simulink model "DynKynValidation"  (R2026b)
settings: Solver=ode5  StopTime=6049.5  FixedStep=1
values from neighbouring files (symbols this model uses):
  A_surf = [Ly*Lz; Lx*Lz; Lx*Ly; Ly*Lz; Lx*Lz; Lx*Ly;            A_panel; A_panel; A_panel; A_panel]    [ValidationAirDrag.m]
  e = e0    (= 0.001)    [ValidationAirDrag.m]    (also in max_disturbance.m = 0.0011)
  i_inc = deg2rad(97.7)    [ValidationAirDrag.m]
  n = sqrt(mu_earth/R^3)    [ValidationAirDrag.m]
  N_surf = [1 0 0; 0 1 0; 0 0 1; -1 0 0; 0 -1 0; 0 0 -1;            1 0 0; -1 0 0; 1 0 0; -1 0 0]    [ValidationAirDrag.m]
  r_CM = r_CM0    [ValidationAirDrag.m]
  R_CP_geom = [Lx/2 0 0; 0 Ly/2 0; 0 0 Lz/2;              -Lx/2 0 0; 0 -Ly/2 0; 0 0 -Lz/2;               0 d_panel 0; 0 d_panel 0; 0 -d_panel 0; 0 -d_panel 0]'    [ValidationAirDrag.m]
undefined symbols (not defined in the file or in its folder): a, angles0, Cd, ecc, hr, I, I_inv, incl, J, rho_atm, true_anomaly_0, w_earth, wB0
libraries: matrix_library x2
settings Model: Creator=39333  LastModifiedBy=enea

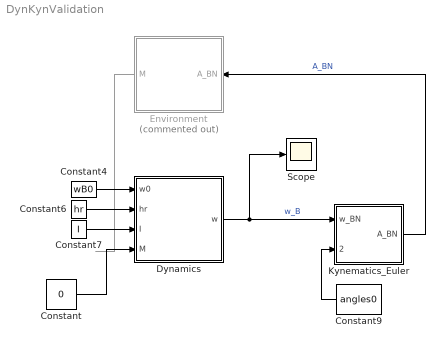
== system DynKynValidation ==
  Constant : Constant  Value=0
  Constant4 : Constant  Value=wB0
  Constant6 : Constant  Value=hr
  Constant7 : Constant  Value=I
  Constant9 : Constant  Value=angles0
  Dynamics : Subsystem
  Environment : Subsystem  Commented=on
  Kynematics_Euler : Subsystem
  Scope : Scope
      settings: ActiveDisplayYMinimum=-0.28630791111671289  ActiveDisplayYMaximum=1.1434373830960349  DataLoggingVariableName=ScopeData2
  wires:
  Constant9/1 -> Kynematics_Euler/2(angles0)
  Kynematics_Euler/1(A_BN) -> Environment/1(A_BN)  "A_BN"
  Environment/1(M) -> ?
  Constant7/1 -> Dynamics/3(I)
  Constant6/1 -> Dynamics/2(hr)
  Constant/1 -> Dynamics/4(M)
  Constant4/1 -> Dynamics/1(w0)
  Dynamics/1(w) -> Scope/1, Kynematics_Euler/1(w_BN)  "w_B"

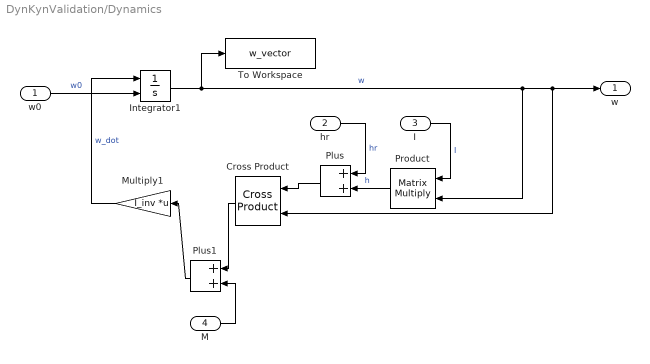
== system DynKynValidation/Dynamics ==
  w0 : Inport
  hr : Inport  Port=2
  I : Inport  Port=3
  M : Inport  Port=4
  Cross Product : matrix_library/Cross Product
  Integrator1 : Integrator  InitialConditionSource=external
  Multiply1 : Gain  Gain=I_inv  Multiplication=Matrix(K*u)
  Plus : Sum
  Plus1 : Sum
  Product : Product  Multiplication=Matrix(*)
  To Workspace : ToWorkspace  VariableName=w_vector  SampleTime=-1
  w : Outport
  wires:
  M/1 -> Plus1/2
  Plus1/1 -> Multiply1/1
  Cross Product/1 -> Plus1/1
  Multiply1/1 -> Integrator1/1  "w_dot"
  I/1 -> Product/1  "I"
  Plus/1 -> Cross Product/1
  Product/1 -> Plus/2  "h"
  Integrator1/1 -> Product/2, Cross Product/2, w/1, To Workspace/1  "w"
  w0/1 -> Integrator1/2  "w0"
  hr/1 -> Plus/1  "hr"

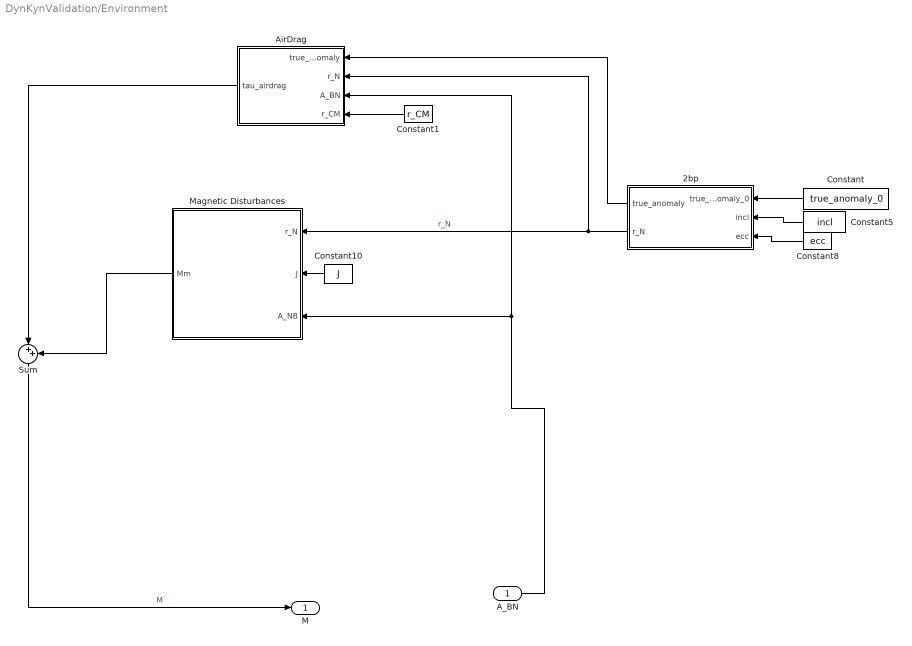
== system DynKynValidation/Environment ==
  A_BN : Inport
  2bp : Subsystem
  AirDrag : Subsystem
  Constant : Constant  Value=true_anomaly_0
  Constant1 : Constant  Value=r_CM
  Constant10 : Constant  Value=J
  Constant5 : Constant  Value=incl
  Constant8 : Constant  Value=ecc
  Magnetic Disturbances : Subsystem
  Sum : Sum  Inputs=|++
  M : Outport
  wires:
  2bp/2(r_N) -> AirDrag/2(r_N), Magnetic Disturbances/1(r_N)  "r_N"
  Magnetic Disturbances/1(Mm) -> Sum/2
  Constant1/1 -> AirDrag/4(r_CM)
  AirDrag/1(tau_airdrag) -> Sum/1
  Constant/1 -> 2bp/1(true_anomaly_0)
  2bp/1(true_anomaly) -> AirDrag/1(true_anomaly)
  Constant5/1 -> 2bp/2(incl)
  Constant10/1 -> Magnetic Disturbances/2(J)
  Constant8/1 -> 2bp/3(ecc)
  A_BN/1 -> AirDrag/3(A_BN), Magnetic Disturbances/3(A_NB)
  Sum/1 -> M/1  "M"

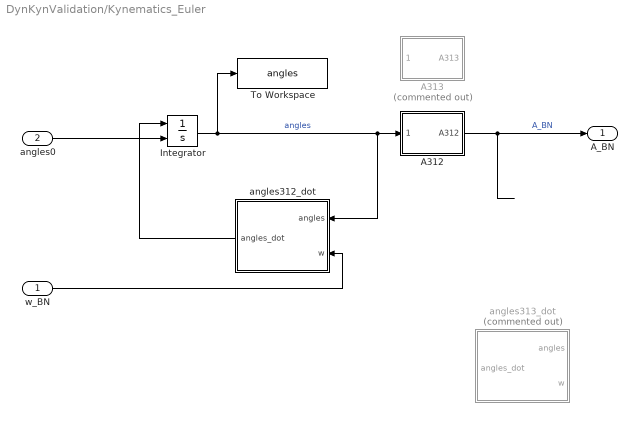
== system DynKynValidation/Kynematics_Euler ==
  w_BN : Inport
  angles0 : Inport  Port=2
  A312 : Subsystem
  A313 : Subsystem  Commented=on
  Integrator : Integrator  InitialConditionSource=external
  To Workspace : ToWorkspace  VariableName=angles  SampleTime=-1
  angles312_dot : Subsystem
  angles313_dot : Subsystem  Commented=on
  A_BN : Outport
  wires:
  Integrator/1 -> A312/1(angles), angles312_dot/1(angles), To Workspace/1  "angles"
  A312/1(A312) -> A_BN/1  "A_BN"
  angles0/1 -> Integrator/2
  angles312_dot/1(angles_dot) -> Integrator/1
  w_BN/1 -> angles312_dot/2(w)

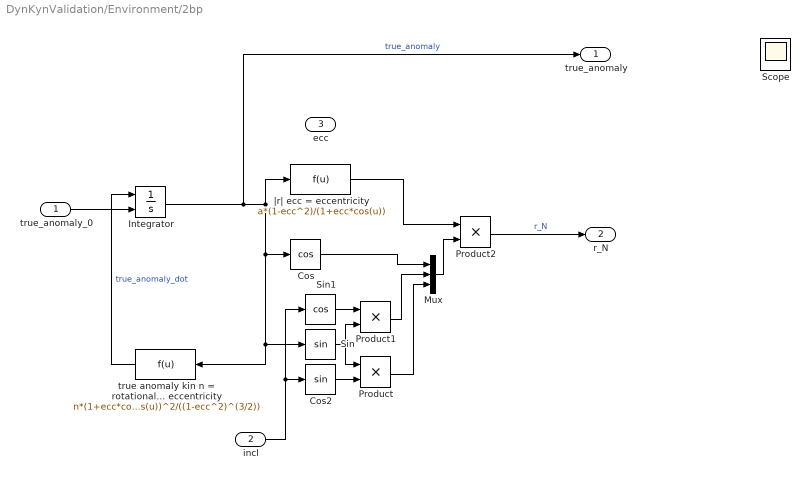
== system DynKynValidation/Environment/2bp ==
  true_anomaly_0 : Inport
  incl : Inport  Port=2
  ecc : Inport  Port=3
  Cos : Trigonometry  Operator=cos
  Cos2 : Trigonometry
  Integrator : Integrator  InitialConditionSource=external
  Mux : Mux  Inputs=3
  Product : Product
  Product1 : Product
  Product2 : Product
  Scope : Scope
  Sin : Trigonometry
  Sin1 : Trigonometry  Operator=cos
  "true anomaly kin n = rotational rate ecc = eccentricity " : Fcn  Expr=n*(1+ecc*cos(u))^2/((1-ecc^2)^(3/2))
  |r| ecc = eccentricity : Fcn  Expr=a*(1-ecc^2)/(1+ecc*cos(u))
  true_anomaly : Outport
  r_N : Outport  Port=2
  wires:
  Sin1/1 -> Product1/1
  Product/1 -> Mux/3
  |r| ecc = eccentricity/1 -> Product2/1
  Cos/1 -> Mux/1
  Product1/1 -> Mux/2
  Integrator/1 -> true_anomaly/1, |r| ecc = eccentricity/1, Sin/1, "true anomaly kin n = rotational rate ecc = eccentricity "/1, Cos/1  "true_anomaly"
  Mux/1 -> Product2/2
  Product2/1 -> r_N/1  "r_N"
  Sin/1 -> Product1/2, Product/1
  "true anomaly kin n = rotational rate ecc = eccentricity "/1 -> Integrator/1  "true_anomaly_dot"
  true_anomaly_0/1 -> Integrator/2
  incl/1 -> Cos2/1, Sin1/1
  Cos2/1 -> Product/2

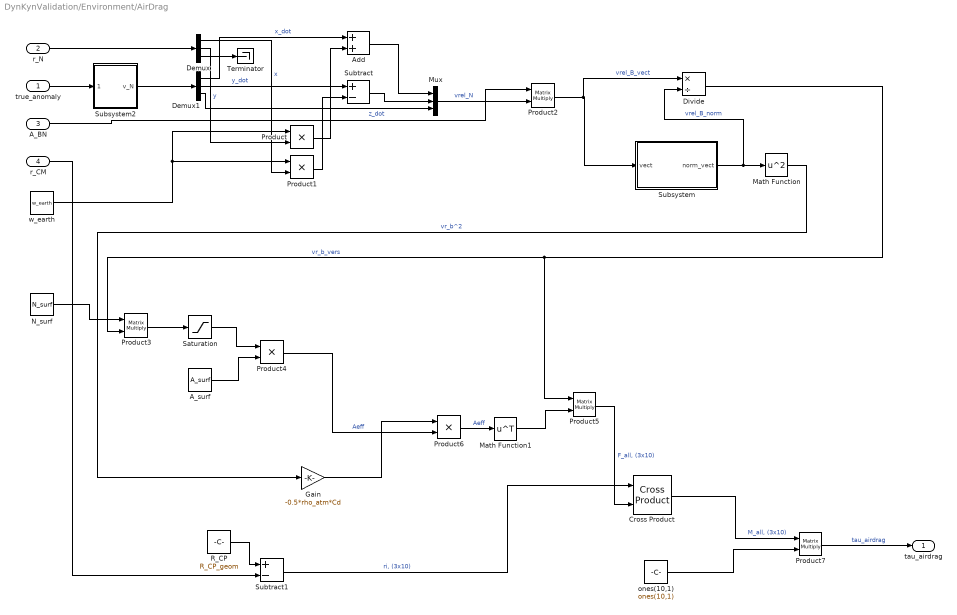
== system DynKynValidation/Environment/AirDrag ==
  true_anomaly : Inport
  r_N : Inport  Port=2
  A_BN : Inport  Port=3
  r_CM : Inport  Port=4
  A_surf : Constant  Value=A_surf
  Add : Sum
  Cross Product : matrix_library/Cross Product
  Demux : Demux  Outputs=3
  Demux1 : Demux  Outputs=3
  Divide : Product  Inputs=*/
  Gain : Gain  Gain=-0.5*rho_atm*Cd
  Math Function : Math  Operator=square
  Math Function1 : Math  Operator=transpose
  Mux : Mux  Inputs=3
  N_surf : Constant  Value=N_surf
  Product{,1,4,6} (4 alike) : Product
  Product{2..3,5,7} (4 alike) : Product  Multiplication=Matrix(*)
  R_CP : Constant  Value=R_CP_geom
  Saturation : Saturate  UpperLimit=inf  LowerLimit=0
  Subsystem : Subsystem
  Subsystem2 : Subsystem
  Subtract : Sum  Inputs=+-
  Subtract1 : Sum  Inputs=+-
  Terminator : Terminator
  ones(10,1) : Constant  Value=ones(10,1)
  w_earth : Constant  Value=w_earth
  tau_airdrag : Outport
  wires:
  Divide/1 -> Product3/2, Product5/1  "vr_b_vers"
  Product4/1 -> Product6/2  "Aeff"
  w_earth/1 -> Product/1, Product1/1
  Demux/3 -> Terminator/1
  Math Function1/1 -> Product5/2
  Demux/2 -> Product/2  "y"
  Demux1/2 -> Subtract/1  "y_dot"
  Demux/1 -> Product1/2  "x"
  Product6/1 -> Math Function1/1  "Aeff"
  Product2/1 -> Divide/1, Subsystem/1(vect)  "vrel_B_vect"
  Gain/1 -> Product6/1
  Add/1 -> Mux/1
  Cross Product/1 -> Product7/1  "M_all, (3x10)"
  Demux1/1 -> Add/1  "x_dot"
  Subsystem2/1(v_N) -> Demux1/1
  Subsystem/1(norm_vect) -> Divide/2, Math Function/1  "vrel_B_norm"
  A_surf/1 -> Product4/2
  Subtract/1 -> Mux/2
  R_CP/1 -> Subtract1/1
  Subtract1/1 -> Cross Product/1  "ri, (3x10)"
  Demux1/3 -> Mux/3  "z_dot"
  Product/1 -> Add/2
  Mux/1 -> Product2/2  "vrel_N"
  Product3/1 -> Saturation/1
  Saturation/1 -> Product4/1
  A_BN/1 -> Product2/1
  Math Function/1 -> Gain/1  "vr_b^2"
  Product1/1 -> Subtract/2
  N_surf/1 -> Product3/1
  Product7/1 -> tau_airdrag/1  "tau_airdrag"
  ones(10,1)/1 -> Product7/2
  Product5/1 -> Cross Product/2  "F_all, (3x10)"
  r_N/1 -> Demux/1
  true_anomaly/1 -> Subsystem2/1(true_anomaly)
  r_CM/1 -> Subtract1/2

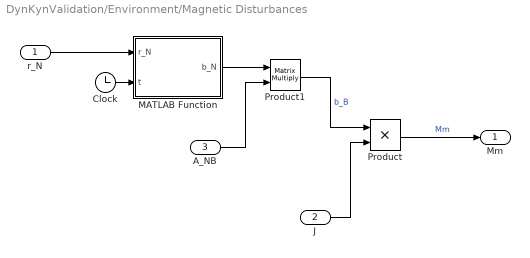
== system DynKynValidation/Environment/Magnetic Disturbances ==
  r_N : Inport
  J : Inport  Port=2
  A_NB : Inport  Port=3
  Clock : Clock
  MATLAB Function : MATLAB Function  TreatAsAtomicUnit=on
  Product : Product
  Product1 : Product  Multiplication=Matrix(*)
  Mm : Outport
  wires:
  Product1/1 -> Product/1  "b_B"
  Clock/1 -> MATLAB Function/2(t)
  MATLAB Function/1(b_N) -> Product1/1
  Product/1 -> Mm/1  "Mm"
  A_NB/1 -> Product1/2
  J/1 -> Product/2
  r_N/1 -> MATLAB Function/1(r_N)

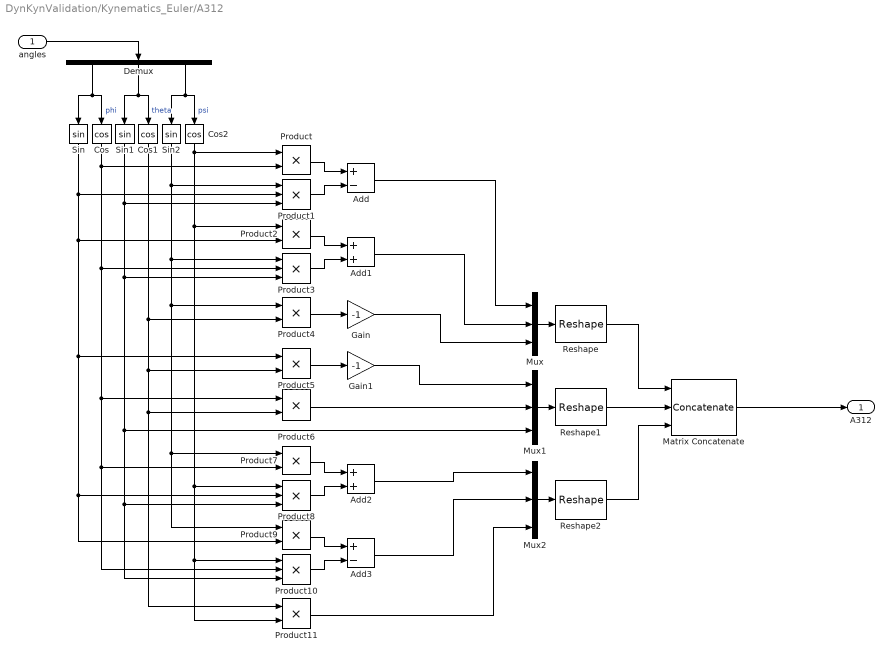
== system DynKynValidation/Kynematics_Euler/A312 ==
  angles : Inport
  Add : Sum  Inputs=+-
  Add1 : Sum
  Add2 : Sum
  Add3 : Sum  Inputs=+-
  Cos : Trigonometry  Operator=cos
  Cos1 : Trigonometry  Operator=cos
  Cos2 : Trigonometry  Operator=cos
  Demux : Demux  Outputs=3
  Gain : Gain  Gain=-1
  Gain1 : Gain  Gain=-1
  Matrix Concatenate : Concatenate  NumInputs=3  Mode=Multidimensional array
  Mux : Mux  Inputs=3
  Mux1 : Mux  Inputs=3
  Mux2 : Mux  Inputs=3
  Product{,2,4..7,9,11} (8 alike) : Product
  Product{1,3,8,10} (4 alike) : Product  Inputs=3
  Reshape : Reshape  OutputDimensionality=Row vector (2-D)  OutputDimensions=[3,1]
  Reshape1 : Reshape  OutputDimensionality=Row vector (2-D)  OutputDimensions=[3,1]
  Reshape2 : Reshape  OutputDimensionality=Row vector (2-D)  OutputDimensions=[3,1]
  Sin : Trigonometry
  Sin1 : Trigonometry
  Sin2 : Trigonometry
  A312 : Outport
  wires:
  Add3/1 -> Mux2/2
  Sin/1 -> Product2/2, Product9/2, Product8/2, Product5/1, Product1/2
  Add1/1 -> Mux/2
  Demux/2 -> Cos1/1, Sin1/1  "theta"
  Sin1/1 -> Product10/3, Product8/3, Mux1/3, Product3/3, Product1/3
  Cos2/1 -> Product2/1, Product11/2, Product10/1, Product8/1, Product/1
  Demux/1 -> Cos/1, Sin/1  "phi"
  Cos1/1 -> Product5/2, Product11/1, Product6/2, Product4/2
  Product/1 -> Add/1
  Sin2/1 -> Product4/1, Product7/1, Product9/1, Product3/1, Product1/1
  Gain1/1 -> Mux1/1
  Product4/1 -> Gain/1
  Product11/1 -> Mux2/3
  Cos/1 -> Product10/2, Product7/2, Product6/1, Product3/2, Product/2
  Demux/3 -> Sin2/1, Cos2/1  "psi"
  Product10/1 -> Add3/2
  Product5/1 -> Gain1/1
  Add2/1 -> Mux2/1
  Product7/1 -> Add2/1
  Product3/1 -> Add1/2
  Product8/1 -> Add2/2
  Product9/1 -> Add3/1
  Product1/1 -> Add/2
  Reshape/1 -> Matrix Concatenate/1
  Product6/1 -> Mux1/2
  Gain/1 -> Mux/3
  Add/1 -> Mux/1
  Product2/1 -> Add1/1
  Matrix Concatenate/1 -> A312/1
  Mux2/1 -> Reshape2/1
  Reshape2/1 -> Matrix Concatenate/3
  Reshape1/1 -> Matrix Concatenate/2
  Mux/1 -> Reshape/1
  Mux1/1 -> Reshape1/1
  angles/1 -> Demux/1

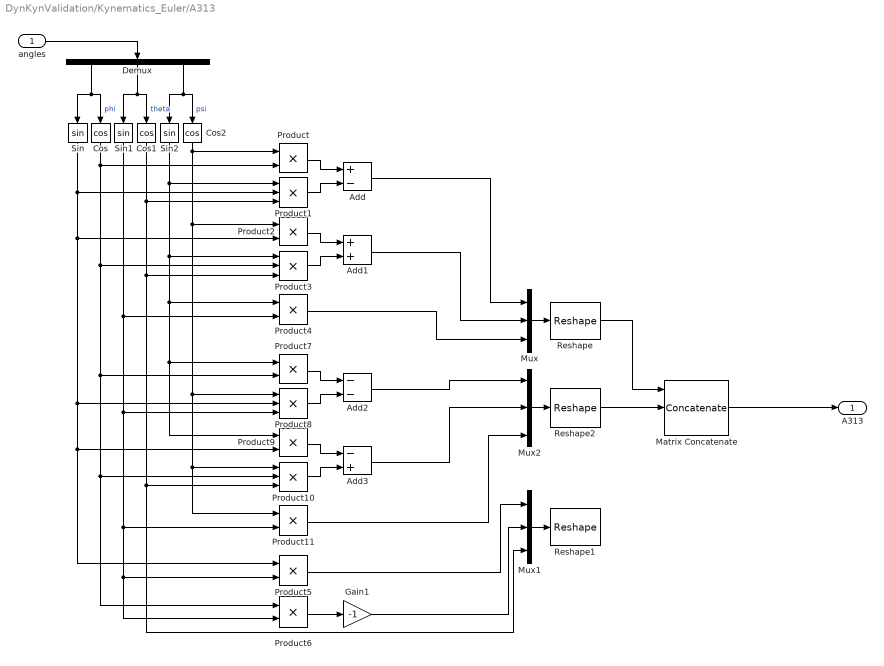
== system DynKynValidation/Kynematics_Euler/A313 ==
  angles : Inport
  Add : Sum  Inputs=+-
  Add1 : Sum
  Add2 : Sum  Inputs=--
  Add3 : Sum  Inputs=-+
  Cos : Trigonometry  Operator=cos
  Cos1 : Trigonometry  Operator=cos
  Cos2 : Trigonometry  Operator=cos
  Demux : Demux  Outputs=3
  Gain1 : Gain  Gain=-1
  Matrix Concatenate : Concatenate  NumInputs=3  Mode=Multidimensional array
  Mux : Mux  Inputs=3
  Mux1 : Mux  Inputs=3
  Mux2 : Mux  Inputs=3
  Product{,2,4..7,9,11} (8 alike) : Product
  Product{1,3,8,10} (4 alike) : Product  Inputs=3
  Reshape : Reshape  OutputDimensionality=Row vector (2-D)  OutputDimensions=[3,1]
  Reshape1 : Reshape  OutputDimensionality=Row vector (2-D)  OutputDimensions=[3,1]
  Reshape2 : Reshape  OutputDimensionality=Row vector (2-D)  OutputDimensions=[3,1]
  Sin : Trigonometry
  Sin1 : Trigonometry
  Sin2 : Trigonometry
  A313 : Outport
  wires:
  Add3/1 -> Mux2/2
  Sin/1 -> Product2/2, Product5/1, Product9/2, Product8/2, Product1/2
  Add1/1 -> Mux/2
  Demux/2 -> Cos1/1, Sin1/1  "theta"
  Sin1/1 -> Product4/2, Product11/2, Product6/2, Product5/2, Product8/3
  Cos2/1 -> Product2/1, Product11/1, Product10/1, Product8/1, Product/1
  Demux/1 -> Cos/1, Sin/1  "phi"
  Cos1/1 -> Product1/3, Product3/3, Mux1/3, Product10/3
  Product/1 -> Add/1
  Sin2/1 -> Product4/1, Product7/1, Product9/1, Product3/1, Product1/1
  Product5/1 -> Mux1/1
  Product11/1 -> Mux2/3
  Cos/1 -> Product6/1, Product10/2, Product7/2, Product3/2, Product/2
  Demux/3 -> Sin2/1, Cos2/1  "psi"
  Product10/1 -> Add3/2
  Add2/1 -> Mux2/1
  Product7/1 -> Add2/1
  Product3/1 -> Add1/2
  Product8/1 -> Add2/2
  Product9/1 -> Add3/1
  Product1/1 -> Add/2
  Reshape/1 -> Matrix Concatenate/1
  Product6/1 -> Gain1/1
  Product4/1 -> Mux/3
  Add/1 -> Mux/1
  Product2/1 -> Add1/1
  Matrix Concatenate/1 -> A313/1
  Mux2/1 -> Reshape2/1
  Mux/1 -> Reshape/1
  Mux1/1 -> Reshape1/1
  angles/1 -> Demux/1
  Reshape2/1 -> Matrix Concatenate/2
  Gain1/1 -> Mux1/2

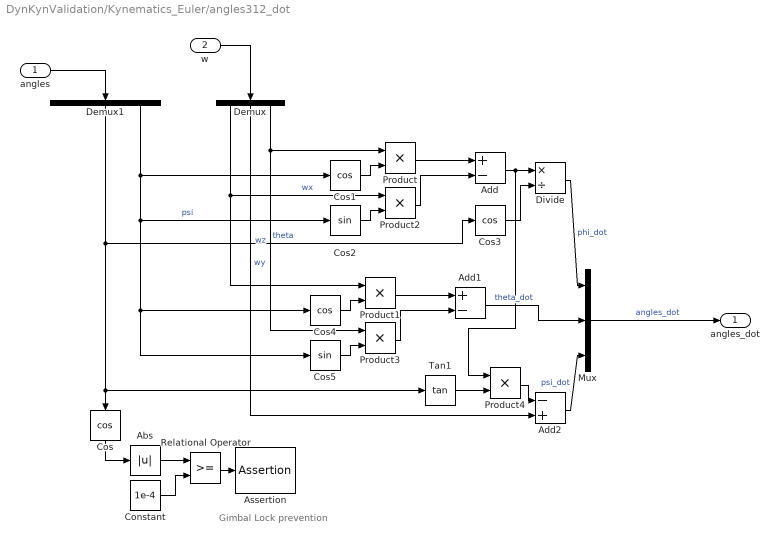
== system DynKynValidation/Kynematics_Euler/angles312_dot ==
  note: Gimbal Lock prevention
  angles : Inport
  w : Inport  Port=2
  Abs : Abs  SaturateOnIntegerOverflow=off
  Add : Sum  Inputs=+-
  Add1 : Sum  Inputs=+-
  Add2 : Sum  Inputs=-+
  Assertion : Assertion  AssertionFailFcn='Gimbal Lock Detected'  StopWhenAssertionFail=off
  Constant : Constant  Value=1e-4
  Cos{,1,3..4} (4 alike) : Trigonometry  Operator=cos
  Cos2 : Trigonometry
  Cos5 : Trigonometry
  Demux : Demux  Outputs=3
  Demux1 : Demux  Outputs=3
  Divide : Product  Inputs=*/
  Mux : Mux  Inputs=3
  Product{,1..4} (5 alike) : Product
  Relational Operator : RelationalOperator  OutDataTypeStr=boolean  RndMeth=Simplest  InputSameDT=off
  Tan1 : Trigonometry  Operator=tan
  angles_dot : Outport
  wires:
  Cos5/1 -> Product3/2
  Add/1 -> Product4/1, Divide/1
  Cos2/1 -> Product2/2
  Demux1/3 -> Cos1/1, Cos2/1, Cos4/1, Cos5/1  "psi"
  Demux1/2 -> Cos/1, Tan1/1, Cos3/1  "theta"
  Cos4/1 -> Product1/2
  Cos1/1 -> Product/2
  Demux/3 -> Product3/1, Product/1  "wz"
  Demux/1 -> Product1/1, Product2/1  "wx"
  Product/1 -> Add/1
  Tan1/1 -> Product4/2
  w/1 -> Demux/1
  Divide/1 -> Mux/1  "phi_dot"
  Cos3/1 -> Divide/2
  Product2/1 -> Add/2
  Product3/1 -> Add1/2
  Product1/1 -> Add1/1
  Add1/1 -> Mux/2  "theta_dot"
  Mux/1 -> angles_dot/1  "angles_dot"
  Product4/1 -> Add2/1
  Add2/1 -> Mux/3  "psi_dot"
  Demux/2 -> Add2/2  "wy"
  angles/1 -> Demux1/1
  Relational Operator/1 -> Assertion/1
  Constant/1 -> Relational Operator/2
  Abs/1 -> Relational Operator/1
  Cos/1 -> Abs/1

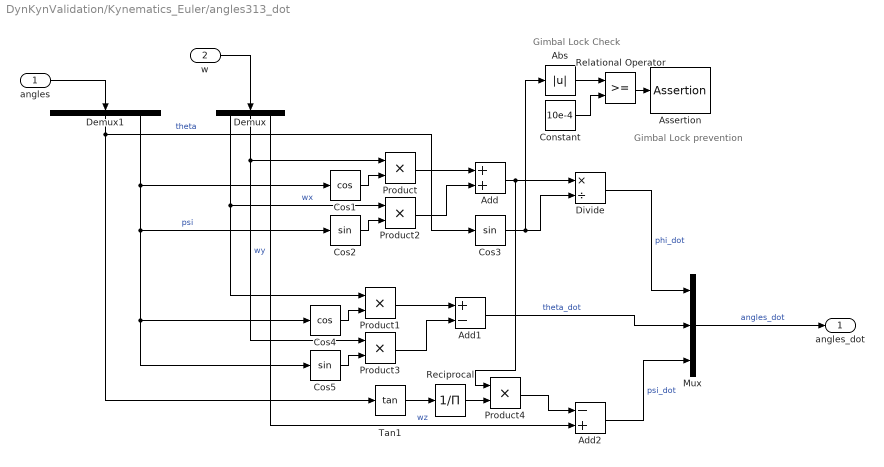
== system DynKynValidation/Kynematics_Euler/angles313_dot ==
  note: Gimbal Lock Check
  note: Gimbal Lock prevention
  angles : Inport
  w : Inport  Port=2
  Abs : Abs  SaturateOnIntegerOverflow=off
  Add : Sum
  Add1 : Sum  Inputs=+-
  Add2 : Sum  Inputs=-+
  Assertion : Assertion  AssertionFailFcn='Gimbal Lock Detected'  StopWhenAssertionFail=off
  Constant : Constant  Value=10e-4
  Cos1 : Trigonometry  Operator=cos
  Cos2 : Trigonometry
  Cos3 : Trigonometry
  Cos4 : Trigonometry  Operator=cos
  Cos5 : Trigonometry
  Demux : Demux  Outputs=3
  Demux1 : Demux  Outputs=3
  Divide : Product  Inputs=*/
  Mux : Mux  Inputs=3
  Product{,1..4} (5 alike) : Product
  Reciprocal : Product  Inputs=/
  Relational Operator : RelationalOperator  OutDataTypeStr=boolean  RndMeth=Simplest  InputSameDT=off
  Tan1 : Trigonometry  Operator=tan
  angles_dot : Outport
  wires:
  Cos5/1 -> Product3/2
  Add/1 -> Product4/1, Divide/1
  Cos2/1 -> Product2/2
  Demux1/3 -> Cos4/1, Cos5/1, Cos2/1, Cos1/1  "psi"
  Demux1/2 -> Tan1/1, Cos3/1  "theta"
  Cos4/1 -> Product1/2
  Cos1/1 -> Product/2
  Demux/1 -> Product1/1, Product2/1  "wx"
  Product/1 -> Add/1
  Tan1/1 -> Reciprocal/1
  w/1 -> Demux/1
  Divide/1 -> Mux/1  "phi_dot"
  Product2/1 -> Add/2
  Product3/1 -> Add1/2
  Product1/1 -> Add1/1
  Add1/1 -> Mux/2  "theta_dot"
  Mux/1 -> angles_dot/1  "angles_dot"
  Product4/1 -> Add2/1
  Add2/1 -> Mux/3  "psi_dot"
  Demux/2 -> Product/1, Product3/1  "wy"
  angles/1 -> Demux1/1
  Demux/3 -> Add2/2  "wz"
  Reciprocal/1 -> Product4/2
  Cos3/1 -> Abs/1, Divide/2
  Relational Operator/1 -> Assertion/1
  Abs/1 -> Relational Operator/1
  Constant/1 -> Relational Operator/2

== system DynKynValidation/Environment/AirDrag/Subsystem ==
  vect : Inport
  Add1 : Sum  Inputs=+++
  Demux2 : Demux  Outputs=3
  Math Function : Math  Operator=square
  Math Function1 : Math  Operator=square
  Math Function2 : Math  Operator=square
  Sqrt : Sqrt
  norm_vect : Outport
  wires:
  Math Function1/1 -> Add1/2
  Math Function2/1 -> Add1/3
  Demux2/2 -> Math Function1/1
  Math Function/1 -> Add1/1
  vect/1 -> Demux2/1
  Demux2/3 -> Math Function2/1
  Demux2/1 -> Math Function/1
  Add1/1 -> Sqrt/1
  Sqrt/1 -> norm_vect/1  "norm_vect"

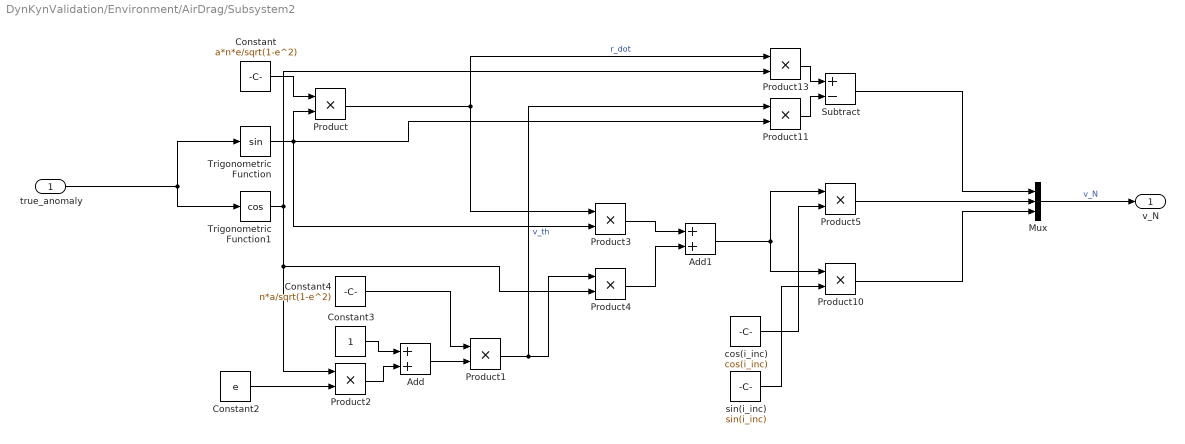
== system DynKynValidation/Environment/AirDrag/Subsystem2 ==
  true_anomaly : Inport
  Add : Sum
  Add1 : Sum
  Constant : Constant  Value=a*n*e/sqrt(1-e^2)
  Constant2 : Constant  Value=e
  Constant3 : Constant
  Constant4 : Constant  Value=n*a/sqrt(1-e^2)
  Mux : Mux  Inputs=3
  Product{,1..5,10..11,13} (9 alike) : Product
  Subtract : Sum  Inputs=+-
  Trigonometric Function : Trigonometry
  Trigonometric Function1 : Trigonometry  Operator=cos
  cos(i_inc) : Constant  Value=cos(i_inc)
  sin(i_inc) : Constant  Value=sin(i_inc)
  v_N : Outport
  wires:
  Constant/1 -> Product/1
  Subtract/1 -> Mux/1
  Product1/1 -> Product11/1, Product4/1  "v_th"
  Product13/1 -> Subtract/1
  Trigonometric Function/1 -> Product11/2, Product3/2, Product/2
  Product4/1 -> Add1/2
  Trigonometric Function1/1 -> Product4/2, Product2/1, Product13/2
  true_anomaly/1 -> Trigonometric Function/1, Trigonometric Function1/1
  Product2/1 -> Add/2
  Product/1 -> Product3/1, Product13/1  "r_dot"
  sin(i_inc)/1 -> Product10/2
  Constant4/1 -> Product1/1
  Product3/1 -> Add1/1
  Add1/1 -> Product5/1, Product10/1
  cos(i_inc)/1 -> Product5/2
  Product5/1 -> Mux/2
  Constant2/1 -> Product2/2
  Add/1 -> Product1/2
  Product10/1 -> Mux/3
  Constant3/1 -> Add/1
  Product11/1 -> Subtract/2
  Mux/1 -> v_N/1  "v_N"

== matlab function DynKynValidation/Environment/Magnetic Disturbances/MATLAB Function ==
  data: r_N input; b_N output; t input
function b_N = magnetic(r_N, t)

% Constants
R_earth = 6371.2; % [km] 
omega_earth = 7.292115e-5; % [rad/s]
alpha_G0 = 0;
k = 10;

% Matrix Preallocation
g = zeros(11, 11);
h = zeros(11, 11);
S = zeros(11, 11);
P = zeros(11, 11);
dP = zeros(11, 11);

% IGRF-13 Epoch 2020.0 Schmidt coefficients in [nT] (index = n+1, m+1)
% taken from https://www.ngdc.noaa.gov/IAGA/vmod/coeffs/igrf13coeffs.txt

% n = 1
g(2, 1) = -29404.8;
g(2, 2) =  -1450.9;  h(2, 2) =  4652.5;

% n = 2
g(3, 1) =  -2499.6;
g(3, 2) =   2982.0;  h(3, 2) = -2991.6;
g(3, 3) =   1677.0;  h(3, 3) =  -734.6;

% n = 3
g(4, 1) =   1363.2;
g(4, 2) =  -2381.2;  h(4, 2) =   -82.1;
g(4, 3) =   1236.2;  h(4, 3) =   241.9;
g(4, 4) =    525.7;  h(4, 4) =  -543.4;

% n = 4
g(5, 1) =    903.0;
g(5, 2) =    809.5;  h(5, 2) =   281.9;
g(5, 3) =     86.3;  h(5, 3) =  -158.4;
g(5, 4) =   -309.4;  h(5, 4) =   199.7;
g(5, 5) =     48.0;  h(5, 5) =  -349.7;

% n = 5
g(6, 1) =   -234.3;
g(6, 2) =    363.2;  h(6, 2) =     47.7;
g(6, 3) =    187.8;  h(6, 3) =    208.3;
g(6, 4) =   -140.7;  h(6, 4) =   -121.2;
g(6, 5) =   -151.2;  h(6, 5) =     32.3;
g(6, 6) =     13.5;  h(6, 6) =     98.9;

% n = 6
g(7, 1) =     66.0;
g(7, 2) =     65.5;  h(7, 2) =    -19.1;
g(7, 3) =     72.9;  h(7, 3) =     25.1;
g(7, 4) =   -121.5;  h(7, 4) =     52.8;
g(7, 5) =    -36.2;  h(7, 5) =    -64.5;
g(7, 6) =     13.5;  h(7, 6) =      8.9;
g(7, 7) =    -64.7;  h(7, 7) =     68.1;

% n = 7
g(8, 1) =     80.6;
g(8, 2) =    -76.7;  h(8, 2) =    -51.5;
g(8, 3) =     -8.2;  h(8, 3) =    -16.9;
g(8, 4) =     56.5;  h(8, 4) =      2.2;
g(8, 5) =     15.8;  h(8, 5) =     23.5;
g(8, 6) =      6.4;  h(8, 6) =     -2.2;
g(8, 7) =     -7.2;  h(8, 7) =    -27.2;
g(8, 8) =      9.8;  h(8, 8) =     -1.8;

% n = 8
g(9, 1) =     23.7;
g(9, 2) =      9.7;  h(9, 2) =      8.4;
g(9, 3) =    -17.6;  h(9, 3) =    -15.3;
g(9, 4) =     -0.5;  h(9, 4) =     12.8;
g(9, 5) =    -21.1;  h(9, 5) =    -11.7;
g(9, 6) =     15.3;  h(9, 6) =     14.9;
g(9, 7) =     13.7;  h(9, 7) =      3.6;
g(9, 8) =    -16.5;  h(9, 8) =     -6.9;
g(9, 9) =     -0.3;  h(9, 9) =      2.8;

% n = 9
g(10, 1) =     5.0;
g(10, 2) =     8.4;  h(10, 2) =   -23.4;
g(10, 3) =     2.9;  h(10, 3) =    11.0;
g(10, 4) =    -1.5;  h(10, 4) =     9.8;
g(10, 5) =    -1.1;  h(10, 5) =    -5.1;
g(10, 6) =   -13.2;  h(10, 6) =    -6.3;
g(10, 7) =     1.1;  h(10, 7) =     7.8;
g(10, 8) =     8.8;  h(10, 8) =     0.4;
g(10, 9) =    -9.3;  h(10, 9) =    -1.4;
g(10, 10) =  -11.9;  h(10, 10) =    9.6;

% n = 10
g(11, 1) =    -1.9;
g(11, 2) =    -6.2;  h(11, 2) =     3.4;
g(11, 3) =    -0.1;  h(11, 3) =    -0.2;
g(11, 4) =     1.7;  h(11, 4) =     3.6;
g(11, 5) =    -0.9;  h(11, 5) =     4.8;
g(11, 6) =     0.7;  h(11, 6) =    -8.6;
g(11, 7) =    -0.9;  h(11, 7) =    -0.1;
g(11, 8) =     1.9;  h(11, 8) =    -4.3;
g(11, 9) =     1.4;  h(11, 9) =    -3.4;
g(11, 10) =   -2.4;  h(11, 10) =   -0.1;
g(11, 11) =   -3.8;  h(11, 11) =   -8.8;

% Schmidt quasi-normalization to Gaussian normalization (S_{n,m})
S(1, 1) = 1;
for n = 1:k
    S(n+1, 1) = S(n, 1) * (2*n - 1) / n;
    for m = 1:n
        if m == 1
            delta_m1 = 1;
        else
            delta_m1 = 0;
        end
        S(n+1, m+1) = S(n+1, m) * sqrt((delta_m1 + 1) * (n - m + 1) / (n + m));
    end
end

g_norm = S .* g;
h_norm = S .* h;

% --- Spherical coordinates of the satellite ---
x = r_N(1);
y = r_N(2);
z = r_N(3);
r = norm(r_N);

theta = acos(max(-1, min(1, z / r))); % Co-latitude [rad]
delta = pi / 2 - theta;               % Declination [rad]
alpha = atan2(y, x);                  % Right ascension [rad]
alpha_G = alpha_G0 + omega_earth * t; % Greenwich right ascension [rad]
phi = alpha - alpha_G;                % East longitude from Greenwich [rad]

% Associated Legendre Polynomials P_{n,m} and dP_{n,m}/dtheta
sin_theta = sin(theta);
cos_theta = cos(theta);

P(1, 1) = 1;
dP(1, 1) = 0;

for n = 1:k
    % Diagonal terms (m = n)
    P(n+1, n+1) = sin_theta * P(n, n);
    dP(n+1, n+1) = sin_theta * dP(n, n) + cos_theta * P(n, n);

    % Sub-diagonal terms (m = 0 ... n-1)
    for m = 0:(n - 1)
        if n == 1
            P(n+1, m+1) = cos_theta * P(n, m+1);
            dP(n+1, m+1) = cos_theta * dP(n, m+1) - sin_theta * P(n, m+1);
        else
            K = ((n - 1)^2 - m^2) / ((2*n - 1) * (2*n - 3));
            P(n+1, m+1) = cos_theta * P(n, m+1) - K * P(n-1, m+1);
            dP(n+1, m+1) = cos_theta * dP(n, m+1) - sin_theta * P(n, m+1) - K * dP(n-1, m+1);
        end
    end
end

% Spherical magnetic field components (Br, Btheta, Bphi) in [nT]
Br = 0;
Btheta = 0;
Bphi_num = 0;

for n = 1:k
    ratio = (R_earth / r)^(n + 2);
    sum_r = 0;
    sum_theta = 0;
    sum_phi = 0;

    for m = 0:n
        gnm = g_norm(n+1, m+1);
        hnm = h_norm(n+1, m+1);
        cos_mphi = cos(m * phi);
        sin_mphi = sin(m * phi);

        common = gnm * cos_mphi + hnm * sin_mphi;
        sum_r = sum_r + common * P(n+1, m+1);
        sum_theta = sum_theta + common * dP(n+1, m+1);
        sum_phi = sum_phi + m * (-gnm * sin_mphi + hnm * cos_mphi) * P(n+1, m+1);
    end

    Br = Br + ratio * (n + 1) * sum_r;
    Btheta = Btheta - ratio * sum_theta;
    Bphi_num = Bphi_num - ratio * sum_phi;
end

% Check whether 
if abs(sin_theta) < 1e-10 
    sin_theta = 1e-10; 
end
Bphi = Bphi_num / sin_theta;

% Transformation from spherical to geocentric inertial frame [T]
B1 = (Br * cos(delta) + Btheta * sin(delta)) * cos(alpha) - Bphi * sin(alpha);
B2 = (Br * cos(delta) + Btheta * sin(delta)) * sin(alpha) + Bphi * cos(alpha);
B3 =  Br * sin(delta) - Btheta * cos(delta);

b_N = [B1; B2; B3] * 1e-9;
end
